simulink model "rfsoc4x2_ospfb_128"  (R2021a)
(part 14 of 339)

  pol1_in1_last_tap7/1(tap_out) -> adder_1_8/5(din4)
  delay38/1 -> adder_1_8/2(din1)
  delay41/1 -> adder_1_9/1(sync)
  pol1_in1_tap18/4(taps_out) -> delay44/1
  [addr] -> pol1_in1_first_tap8/4(addr_in)
  pol1_in1_first_tap8/6(pot_en_out) -> pol1_in1_tap17/5(pot_en_in)
  pol1_in1_tap17/1(dout) -> pol1_in1_tap18/1(din)
  pol1_in1_tap17/2(sync_out) -> pol1_in1_tap18/2(sync)
  pol1_in1_first_tap8/5(add_out) -> pol1_in1_tap17/4(addr_in)
  pol1_in1_first_tap8/4(taps_out) -> delay42/1
  pol1_in1_tap17/4(taps_out) -> delay43/1
  delay44/1 -> adder_1_9/4(din3)
  pol1_in2_coeffs7/1(dout) -> pol1_in1_first_tap8/1(din)
  [tap_write_en] -> pol1_in1_first_tap8/5(pot_en_in)
  delay43/1 -> adder_1_9/3(din2)
  pol1_in1_first_tap8/3(coeff_out) -> pol1_in1_tap17/3(coeff)
  pol1_in1_last_tap8/2(sync_out) -> delay41/1
  pol1_in2_coeffs7/3(coeff) -> pol1_in1_first_tap8/3(coeffs)
  pol1_in1_tap18/3(coeff_out) -> pol1_in1_last_tap8/3(coeff)
  pol1_in1_tap18/2(sync_out) -> pol1_in1_last_tap8/2(sync)
  pol1_in1_tap17/6(pot_en_out) -> pol1_in1_tap18/5(pot_en_in)
  pol1_in1_tap17/5(add_out) -> pol1_in1_tap18/4(addr_in)
  pol1_in1_tap18/1(dout) -> pol1_in1_last_tap8/1(din)
  pol1_in1_first_tap8/2(sync_out) -> pol1_in1_tap17/2(sync)
  pol1_in1_tap17/3(coeff_out) -> pol1_in1_tap18/3(coeff)
  pol1_in2_coeffs7/2(sync_out) -> pol1_in1_first_tap8/2(sync)
  pol1_in1_first_tap8/1(dout) -> pol1_in1_tap17/1(din)
  pol1_in1_last_tap8/1(tap_out) -> adder_1_9/5(din4)
  delay42/1 -> adder_1_9/2(din1)
  delay45/1 -> adder_1_10/1(sync)
  pol1_in1_tap20/4(taps_out) -> delay48/1
  [addr] -> pol1_in1_first_tap9/4(addr_in)
  pol1_in1_first_tap9/6(pot_en_out) -> pol1_in1_tap19/5(pot_en_in)
  pol1_in1_tap19/1(dout) -> pol1_in1_tap20/1(din)
  pol1_in1_tap19/2(sync_out) -> pol1_in1_tap20/2(sync)
  pol1_in1_first_tap9/5(add_out) -> pol1_in1_tap19/4(addr_in)
  pol1_in1_first_tap9/4(taps_out) -> delay46/1
  pol1_in1_tap19/4(taps_out) -> delay47/1
  delay48/1 -> adder_1_10/4(din3)
  pol1_in2_coeffs8/1(dout) -> pol1_in1_first_tap9/1(din)
  [tap_write_en] -> pol1_in1_first_tap9/5(pot_en_in)
  delay47/1 -> adder_1_10/3(din2)
  pol1_in1_first_tap9/3(coeff_out) -> pol1_in1_tap19/3(coeff)
  pol1_in1_last_tap9/2(sync_out) -> delay45/1
  pol1_in2_coeffs8/3(coeff) -> pol1_in1_first_tap9/3(coeffs)
  pol1_in1_tap20/3(coeff_out) -> pol1_in1_last_tap9/3(coeff)
  pol1_in1_tap20/2(sync_out) -> pol1_in1_last_tap9/2(sync)
  pol1_in1_tap19/6(pot_en_out) -> pol1_in1_tap20/5(pot_en_in)
  pol1_in1_tap19/5(add_out) -> pol1_in1_tap20/4(addr_in)
  pol1_in1_tap20/1(dout) -> pol1_in1_last_tap9/1(din)
  pol1_in1_first_tap9/2(sync_out) -> pol1_in1_tap19/2(sync)
  pol1_in1_tap19/3(coeff_out) -> pol1_in1_tap20/3(coeff)
  pol1_in2_coeffs8/2(sync_out) -> pol1_in1_first_tap9/2(sync)
  pol1_in1_first_tap9/1(dout) -> pol1_in1_tap19/1(din)
  pol1_in1_last_tap9/1(tap_out) -> adder_1_10/5(din4)
  delay46/1 -> adder_1_10/2(din1)
  delay49/1 -> adder_1_11/1(sync)
  pol1_in1_tap22/4(taps_out) -> delay52/1
  [addr] -> pol1_in1_first_tap10/4(addr_in)
  pol1_in1_first_tap10/6(pot_en_out) -> pol1_in1_tap21/5(pot_en_in)
  pol1_in1_tap21/1(dout) -> pol1_in1_tap22/1(din)
  pol1_in1_tap21/2(sync_out) -> pol1_in1_tap22/2(sync)
  pol1_in1_first_tap10/5(add_out) -> pol1_in1_tap21/4(addr_in)
  pol1_in1_first_tap10/4(taps_out) -> delay50/1
  pol1_in1_tap21/4(taps_out) -> delay51/1
  delay52/1 -> adder_1_11/4(din3)
  pol1_in2_coeffs9/1(dout) -> pol1_in1_first_tap10/1(din)
  [tap_write_en] -> pol1_in1_first_tap10/5(pot_en_in)
  delay51/1 -> adder_1_11/3(din2)
  pol1_in1_first_tap10/3(coeff_out) -> pol1_in1_tap21/3(coeff)
  pol1_in1_last_tap10/2(sync_out) -> delay49/1
  pol1_in2_coeffs9/3(coeff) -> pol1_in1_first_tap10/3(coeffs)
  pol1_in1_tap22/3(coeff_out) -> pol1_in1_last_tap10/3(coeff)
  pol1_in1_tap22/2(sync_out) -> pol1_in1_last_tap10/2(sync)
  pol1_in1_tap21/6(pot_en_out) -> pol1_in1_tap22/5(pot_en_in)
  pol1_in1_tap21/5(add_out) -> pol1_in1_tap22/4(addr_in)
  pol1_in1_tap22/1(dout) -> pol1_in1_last_tap10/1(din)
  pol1_in1_first_tap10/2(sync_out) -> pol1_in1_tap21/2(sync)
  pol1_in1_tap21/3(coeff_out) -> pol1_in1_tap22/3(coeff)
  pol1_in2_coeffs9/2(sync_out) -> pol1_in1_first_tap10/2(sync)
  pol1_in1_first_tap10/1(dout) -> pol1_in1_tap21/1(din)
  pol1_in1_last_tap10/1(tap_out) -> adder_1_11/5(din4)
  delay50/1 -> adder_1_11/2(din1)
  delay53/1 -> adder_1_12/1(sync)
  pol1_in1_tap24/4(taps_out) -> delay56/1
  [addr] -> pol1_in1_first_tap11/4(addr_in)
  pol1_in1_first_tap11/6(pot_en_out) -> pol1_in1_tap23/5(pot_en_in)
  pol1_in1_tap23/1(dout) -> pol1_in1_tap24/1(din)
  pol1_in1_tap23/2(sync_out) -> pol1_in1_tap24/2(sync)
  pol1_in1_first_tap11/5(add_out) -> pol1_in1_tap23/4(addr_in)
  pol1_in1_first_tap11/4(taps_out) -> delay54/1
  pol1_in1_tap23/4(taps_out) -> delay55/1
  delay56/1 -> adder_1_12/4(din3)
  pol1_in2_coeffs10/1(dout) -> pol1_in1_first_tap11/1(din)
  [tap_write_en] -> pol1_in1_first_tap11/5(pot_en_in)
  delay55/1 -> adder_1_12/3(din2)
  pol1_in1_first_tap11/3(coeff_out) -> pol1_in1_tap23/3(coeff)
  pol1_in1_last_tap11/2(sync_out) -> delay53/1
  pol1_in2_coeffs10/3(coeff) -> pol1_in1_first_tap11/3(coeffs)
  pol1_in1_tap24/3(coeff_out) -> pol1_in1_last_tap11/3(coeff)
  pol1_in1_tap24/2(sync_out) -> pol1_in1_last_tap11/2(sync)
  pol1_in1_tap23/6(pot_en_out) -> pol1_in1_tap24/5(pot_en_in)
  pol1_in1_tap23/5(add_out) -> pol1_in1_tap24/4(addr_in)
  pol1_in1_tap24/1(dout) -> pol1_in1_last_tap11/1(din)
  pol1_in1_first_tap11/2(sync_out) -> pol1_in1_tap23/2(sync)
  pol1_in1_tap23/3(coeff_out) -> pol1_in1_tap24/3(coeff)
  pol1_in2_coeffs10/2(sync_out) -> pol1_in1_first_tap11/2(sync)
  pol1_in1_first_tap11/1(dout) -> pol1_in1_tap23/1(din)
  pol1_in1_last_tap11/1(tap_out) -> adder_1_12/5(din4)
  delay54/1 -> adder_1_12/2(din1)
  delay57/1 -> adder_1_13/1(sync)
  pol1_in1_tap26/4(taps_out) -> delay60/1
  [addr] -> pol1_in1_first_tap12/4(addr_in)
  pol1_in1_first_tap12/6(pot_en_out) -> pol1_in1_tap25/5(pot_en_in)
  pol1_in1_tap25/1(dout) -> pol1_in1_tap26/1(din)
  pol1_in1_tap25/2(sync_out) -> pol1_in1_tap26/2(sync)
  pol1_in1_first_tap12/5(add_out) -> pol1_in1_tap25/4(addr_in)
  pol1_in1_first_tap12/4(taps_out) -> delay58/1
  pol1_in1_tap25/4(taps_out) -> delay59/1
  delay60/1 -> adder_1_13/4(din3)
  pol1_in2_coeffs11/1(dout) -> pol1_in1_first_tap12/1(din)
  [tap_write_en] -> pol1_in1_first_tap12/5(pot_en_in)
  delay59/1 -> adder_1_13/3(din2)
  pol1_in1_first_tap12/3(coeff_out) -> pol1_in1_tap25/3(coeff)
  pol1_in1_last_tap12/2(sync_out) -> delay57/1
  pol1_in2_coeffs11/3(coeff) -> pol1_in1_first_tap12/3(coeffs)
  pol1_in1_tap26/3(coeff_out) -> pol1_in1_last_tap12/3(coeff)
  pol1_in1_tap26/2(sync_out) -> pol1_in1_last_tap12/2(sync)
  pol1_in1_tap25/6(pot_en_out) -> pol1_in1_tap26/5(pot_en_in)
  pol1_in1_tap25/5(add_out) -> pol1_in1_tap26/4(addr_in)
  pol1_in1_tap26/1(dout) -> pol1_in1_last_tap12/1(din)
  pol1_in1_first_tap12/2(sync_out) -> pol1_in1_tap25/2(sync)
  pol1_in1_tap25/3(coeff_out) -> pol1_in1_tap26/3(coeff)
  pol1_in2_coeffs11/2(sync_out) -> pol1_in1_first_tap12/2(sync)
  pol1_in1_first_tap12/1(dout) -> pol1_in1_tap25/1(din)
  pol1_in1_last_tap12/1(tap_out) -> adder_1_13/5(din4)
  delay58/1 -> adder_1_13/2(din1)
  delay61/1 -> adder_1_14/1(sync)
  pol1_in1_tap28/4(taps_out) -> delay64/1
  [addr] -> pol1_in1_first_tap13/4(addr_in)
  pol1_in1_first_tap13/6(pot_en_out) -> pol1_in1_tap27/5(pot_en_in)
  pol1_in1_tap27/1(dout) -> pol1_in1_tap28/1(din)
  pol1_in1_tap27/2(sync_out) -> pol1_in1_tap28/2(sync)
  pol1_in1_first_tap13/5(add_out) -> pol1_in1_tap27/4(addr_in)
  pol1_in1_first_tap13/4(taps_out) -> delay62/1
  pol1_in1_tap27/4(taps_out) -> delay63/1
  delay64/1 -> adder_1_14/4(din3)
  pol1_in2_coeffs12/1(dout) -> pol1_in1_first_tap13/1(din)
  [tap_write_en] -> pol1_in1_first_tap13/5(pot_en_in)
  delay63/1 -> adder_1_14/3(din2)
  pol1_in1_first_tap13/3(coeff_out) -> pol1_in1_tap27/3(coeff)
  pol1_in1_last_tap13/2(sync_out) -> delay61/1
  pol1_in2_coeffs12/3(coeff) -> pol1_in1_first_tap13/3(coeffs)
  pol1_in1_tap28/3(coeff_out) -> pol1_in1_last_tap13/3(coeff)
  pol1_in1_tap28/2(sync_out) -> pol1_in1_last_tap13/2(sync)
  pol1_in1_tap27/6(pot_en_out) -> pol1_in1_tap28/5(pot_en_in)
  pol1_in1_tap27/5(add_out) -> pol1_in1_tap28/4(addr_in)
  pol1_in1_tap28/1(dout) -> pol1_in1_last_tap13/1(din)
  pol1_in1_first_tap13/2(sync_out) -> pol1_in1_tap27/2(sync)
  pol1_in1_tap27/3(coeff_out) -> pol1_in1_tap28/3(coeff)
  pol1_in2_coeffs12/2(sync_out) -> pol1_in1_first_tap13/2(sync)
  pol1_in1_first_tap13/1(dout) -> pol1_in1_tap27/1(din)
  pol1_in1_last_tap13/1(tap_out) -> adder_1_14/5(din4)
  delay62/1 -> adder_1_14/2(din1)
  pol1_in1_tap30/4(taps_out) -> delay68/1
  [addr] -> pol1_in1_first_tap14/4(addr_in)
  pol1_in1_first_tap14/6(pot_en_out) -> pol1_in1_tap29/5(pot_en_in)
  pol1_in1_tap29/1(dout) -> pol1_in1_tap30/1(din)
  pol1_in1_tap29/2(sync_out) -> pol1_in1_tap30/2(sync)
  pol1_in1_first_tap14/5(add_out) -> pol1_in1_tap29/4(addr_in)
  pol1_in1_first_tap14/4(taps_out) -> delay66/1
  pol1_in1_tap29/4(taps_out) -> delay67/1
  delay68/1 -> adder_1_15/4(din3)
  pol1_in2_coeffs13/1(dout) -> pol1_in1_first_tap14/1(din)
  [tap_write_en] -> pol1_in1_first_tap14/5(pot_en_in)
  delay67/1 -> adder_1_15/3(din2)
  pol1_in1_first_tap14/3(coeff_out) -> pol1_in1_tap29/3(coeff)
  pol1_in1_last_tap14/2(sync_out) -> delay65/1
  pol1_in2_coeffs13/3(coeff) -> pol1_in1_first_tap14/3(coeffs)
  pol1_in1_tap30/3(coeff_out) -> pol1_in1_last_tap14/3(coeff)
  pol1_in1_tap30/2(sync_out) -> pol1_in1_last_tap14/2(sync)
  pol1_in1_tap29/6(pot_en_out) -> pol1_in1_tap30/5(pot_en_in)
  pol1_in1_tap29/5(add_out) -> pol1_in1_tap30/4(addr_in)
  pol1_in1_tap30/1(dout) -> pol1_in1_last_tap14/1(din)
  pol1_in1_first_tap14/2(sync_out) -> pol1_in1_tap29/2(sync)
  pol1_in1_tap29/3(coeff_out) -> pol1_in1_tap30/3(coeff)
  pol1_in2_coeffs13/2(sync_out) -> pol1_in1_first_tap14/2(sync)
  pol1_in1_first_tap14/1(dout) -> pol1_in1_tap29/1(din)
  pol1_in1_last_tap14/1(tap_out) -> adder_1_15/5(din4)
  delay66/1 -> adder_1_15/2(din1)
  delay65/1 -> adder_1_15/1(sync)
  delay69/1 -> adder_1_16/1(sync)
  pol1_in1_tap32/4(taps_out) -> delay72/1
  [addr] -> pol1_in1_first_tap15/4(addr_in)
  pol1_in1_first_tap15/6(pot_en_out) -> pol1_in1_tap31/5(pot_en_in)
  pol1_in1_tap31/1(dout) -> pol1_in1_tap32/1(din)
  pol1_in1_tap31/2(sync_out) -> pol1_in1_tap32/2(sync)
  pol1_in1_first_tap15/5(add_out) -> pol1_in1_tap31/4(addr_in)
  pol1_in1_first_tap15/4(taps_out) -> delay70/1
  pol1_in1_tap31/4(taps_out) -> delay71/1
  delay72/1 -> adder_1_16/4(din3)
  pol1_in2_coeffs14/1(dout) -> pol1_in1_first_tap15/1(din)
  [tap_write_en] -> pol1_in1_first_tap15/5(pot_en_in)
  delay71/1 -> adder_1_16/3(din2)
  pol1_in1_first_tap15/3(coeff_out) -> pol1_in1_tap31/3(coeff)
  pol1_in1_last_tap15/2(sync_out) -> delay69/1
  pol1_in2_coeffs14/3(coeff) -> pol1_in1_first_tap15/3(coeffs)
  pol1_in1_tap32/3(coeff_out) -> pol1_in1_last_tap15/3(coeff)
  pol1_in1_tap32/2(sync_out) -> pol1_in1_last_tap15/2(sync)
  pol1_in1_tap31/6(pot_en_out) -> pol1_in1_tap32/5(pot_en_in)
  pol1_in1_tap31/5(add_out) -> pol1_in1_tap32/4(addr_in)
  pol1_in1_tap32/1(dout) -> pol1_in1_last_tap15/1(din)
  pol1_in1_first_tap15/2(sync_out) -> pol1_in1_tap31/2(sync)
  pol1_in1_tap31/3(coeff_out) -> pol1_in1_tap32/3(coeff)
  pol1_in2_coeffs14/2(sync_out) -> pol1_in1_first_tap15/2(sync)
  pol1_in1_first_tap15/1(dout) -> pol1_in1_tap31/1(din)
  pol1_in1_last_tap15/1(tap_out) -> adder_1_16/5(din4)
  delay70/1 -> adder_1_16/2(din1)
